simulink model "Residential_grid8"  (R2026a)
settings: Solver=VariableStepAuto  StopTime=365*24*3600
undefined symbols (not defined in the file): evCharge, load1, load2, load3, load4, load5, Solar, Wind
libraries: fl_lib x139, nesl_utility x68
(part 2 of 3)

== system Residential_grid8/Battery 5 ==
  1-D Lookup Table1 : Lookup_n-D  NumberOfTableDimensions=1  BreakpointsForDimension1=[0;0.0001;0.00025000000000000001;0.00040000000000000002;0.0007000000000000001;0.001;0.0015;0.0023;0.0040000000000000001;0.0060000000000000001;0.007000000000000001;0.0080000000000000002;0.0089999999999999993;0.0094999999999999998;0.0097999999999999997;0.0099500000000000005;0.01]  Table=[0;1;2.7000000000000002;2.9500000000000002;3.1000000000000001;3.2000000000000002;3.2400000000000002;3.2599999999999998;3.2799999999999998;3.2999999999999998;3.3399999999999999;3.3500000000000001;3.3700000000000001;3.3900000000000001;3.4500000000000002;3.6000000000000001;3.8000000000000003]  InternalRulePriority=Speed  RndMeth=Simplest
  Bus Creator : BusCreator  Inputs=3
  Capacitor : fl_lib/Electrical/Electrical Elements/Capacitor  c=3.6e5*C_batt F  r=0 Ohm  g=0 1/Ohm  i_specify=off  i_priority=None  i=0 A  i_nominal_specify=off  i_nominal_value=1  i_nominal_unit=A  v_specify=off  v_priority=None  v=0 V  v_nominal_specify=off  v_nominal_value=1  v_nominal_unit=V  vc_specify=on  vc_priority=High  vc=SOC_Initial/10000 V  vc_nominal_specify=off  vc_nominal_value=1  vc_nominal_unit=V
  Controlled Voltage Source1 : fl_lib/Electrical/Electrical Sources/Controlled Voltage Source
  Current Sensor : fl_lib/Electrical/Electrical Sensors/Current Sensor
  Gain : Gain  Gain=Cell
  Memory : Memory
  PS-Simulink Converter : nesl_utility/PS-Simulink Converter  PhysicalDomain=network_engine_domain  SubClassName=ps_output  LeftPortType=input  RightPortType=output  PseudoPeriodic=off  Frequencies=[]  VectorFormat=inherit  Unit=inherit  AffineConversion=off
  PS-Simulink Converter1 : nesl_utility/PS-Simulink Converter  PhysicalDomain=network_engine_domain  SubClassName=ps_output  LeftPortType=input  RightPortType=output  PseudoPeriodic=off  Frequencies=[]  VectorFormat=inherit  Unit=inherit  AffineConversion=off
  PS-Simulink Converter2 : nesl_utility/PS-Simulink Converter  PhysicalDomain=network_engine_domain  SubClassName=ps_output  LeftPortType=input  RightPortType=output  PseudoPeriodic=off  Frequencies=[]  VectorFormat=inherit  Unit=inherit  AffineConversion=off
  Product1 : Product
  Resistor : fl_lib/Electrical/Electrical Elements/Resistor  R=1e-3*R_int*Cell/C_batt Ohm  i_specify=off  i_priority=None  i=0 A  i_nominal_specify=off  i_nominal_value=1  i_nominal_unit=A  v_specify=off  v_priority=None  v=0 V  v_nominal_specify=off  v_nominal_value=1  v_nominal_unit=V
  Simulink-PS Converter : nesl_utility/Simulink-PS Converter  PhysicalDomain=network_engine_domain  SubClassName=ps_input  LeftPortType=input  RightPortType=output  PseudoPeriodic=off  Frequencies=[]  NoiseDistribution=none  NoiseParameters=[]  Unit=1  AffineConversion=off  FilteringAndDerivatives=provide  SimscapeFilterOrder=1  InputFilterTimeConstant=0.001  UdotUserProvided=0
  Voltage Sensor : fl_lib/Electrical/Electrical Sensors/Voltage Sensor
  Voltage Sensor1 : fl_lib/Electrical/Electrical Sensors/Voltage Sensor
  + : PMIOPort  Side=Right
  - : PMIOPort  Port=2  Side=Right
  Comp. : Outport
  wires:
  PS-Simulink Converter2/1 -> Product1/1, Bus Creator/2  "IBatt"
  PS-Simulink Converter1/1 -> Bus Creator/3, Product1/2  "VBatt"
  Product1/1 -> Bus Creator/1  "Pbatt5"
  Bus Creator/1 -> Comp./1
  PS-Simulink Converter/1 -> 1-D Lookup Table1/1
  Memory/1 -> Simulink-PS Converter/1
  Gain/1 -> Memory/1
  1-D Lookup Table1/1 -> Gain/1
  connections:
  Voltage Sensor/LConn1 -- Controlled Voltage Source1/RConn2 -- Capacitor/LConn1
  Capacitor/RConn1 -- Voltage Sensor/RConn2 -- -/RConn1 -- Voltage Sensor1/RConn2
  Voltage Sensor1/LConn1 -- +/RConn1 -- Current Sensor/RConn2
  Current Sensor/LConn1 -- Resistor/RConn1
  PS-Simulink Converter/LConn1 -- Voltage Sensor/RConn1
  Controlled Voltage Source1/LConn1 -- Resistor/LConn1
  PS-Simulink Converter1/LConn1 -- Voltage Sensor1/RConn1
  PS-Simulink Converter2/LConn1 -- Current Sensor/RConn1
  Simulink-PS Converter/RConn1 -- Controlled Voltage Source1/RConn1

== system Residential_grid8/Cable 0 ==
  Resistor : fl_lib/Electrical/Electrical Elements/Resistor  R=intR/1000*L Ohm  i_specify=off  i_priority=None  i=0 A  i_nominal_specify=off  i_nominal_value=1  i_nominal_unit=A  v_specify=off  v_priority=None  v=0 V  v_nominal_specify=off  v_nominal_value=1  v_nominal_unit=V
  Resistor1 : fl_lib/Electrical/Electrical Elements/Resistor  R=intR/1000*L Ohm  i_specify=off  i_priority=None  i=0 A  i_nominal_specify=off  i_nominal_value=1  i_nominal_unit=A  v_specify=off  v_priority=None  v=0 V  v_nominal_specify=off  v_nominal_value=1  v_nominal_unit=V
  Series RLC Branch1 : PMIOPort  Side=Left
  Series RLC Branch2 : PMIOPort  Port=2  Side=Right
  Series RLC Branch3 : PMIOPort  Port=3  Side=Left
  Series RLC Branch4 : PMIOPort  Port=4  Side=Right
  connections:
  Series RLC Branch3/RConn1 -- Resistor1/LConn1
  Series RLC Branch2/RConn1 -- Resistor/RConn1
  Series RLC Branch1/RConn1 -- Resistor/LConn1
  Series RLC Branch4/RConn1 -- Resistor1/RConn1

== system Residential_grid8/Cable 1 ==
  Resistor : fl_lib/Electrical/Electrical Elements/Resistor  R=intR/1000*L Ohm  i_specify=off  i_priority=None  i=0 A  i_nominal_specify=off  i_nominal_value=1  i_nominal_unit=A  v_specify=off  v_priority=None  v=0 V  v_nominal_specify=off  v_nominal_value=1  v_nominal_unit=V
  Resistor1 : fl_lib/Electrical/Electrical Elements/Resistor  R=intR/1000*L Ohm  i_specify=off  i_priority=None  i=0 A  i_nominal_specify=off  i_nominal_value=1  i_nominal_unit=A  v_specify=off  v_priority=None  v=0 V  v_nominal_specify=off  v_nominal_value=1  v_nominal_unit=V
  Series RLC Branch1 : PMIOPort  Side=Left
  Series RLC Branch2 : PMIOPort  Port=2  Side=Right
  Series RLC Branch3 : PMIOPort  Port=3  Side=Left
  Series RLC Branch4 : PMIOPort  Port=4  Side=Right
  connections:
  Series RLC Branch3/RConn1 -- Resistor1/LConn1
  Series RLC Branch2/RConn1 -- Resistor/RConn1
  Series RLC Branch1/RConn1 -- Resistor/LConn1
  Series RLC Branch4/RConn1 -- Resistor1/RConn1

== system Residential_grid8/Cable 1-1 ==
  Resistor : fl_lib/Electrical/Electrical Elements/Resistor  R=intR/1000*L Ohm  i_specify=off  i_priority=None  i=0 A  i_nominal_specify=off  i_nominal_value=1  i_nominal_unit=A  v_specify=off  v_priority=None  v=0 V  v_nominal_specify=off  v_nominal_value=1  v_nominal_unit=V
  Resistor1 : fl_lib/Electrical/Electrical Elements/Resistor  R=intR/1000*L Ohm  i_specify=off  i_priority=None  i=0 A  i_nominal_specify=off  i_nominal_value=1  i_nominal_unit=A  v_specify=off  v_priority=None  v=0 V  v_nominal_specify=off  v_nominal_value=1  v_nominal_unit=V
  Series RLC Branch1 : PMIOPort  Side=Left
  Series RLC Branch2 : PMIOPort  Port=2  Side=Right
  Series RLC Branch3 : PMIOPort  Port=3  Side=Left
  Series RLC Branch4 : PMIOPort  Port=4  Side=Right
  connections:
  Series RLC Branch3/RConn1 -- Resistor1/LConn1
  Series RLC Branch2/RConn1 -- Resistor/RConn1
  Series RLC Branch1/RConn1 -- Resistor/LConn1
  Series RLC Branch4/RConn1 -- Resistor1/RConn1

== system Residential_grid8/Cable 1-2 ==
  Resistor : fl_lib/Electrical/Electrical Elements/Resistor  R=intR/1000*L Ohm  i_specify=off  i_priority=None  i=0 A  i_nominal_specify=off  i_nominal_value=1  i_nominal_unit=A  v_specify=off  v_priority=None  v=0 V  v_nominal_specify=off  v_nominal_value=1  v_nominal_unit=V
  Resistor1 : fl_lib/Electrical/Electrical Elements/Resistor  R=intR/1000*L Ohm  i_specify=off  i_priority=None  i=0 A  i_nominal_specify=off  i_nominal_value=1  i_nominal_unit=A  v_specify=off  v_priority=None  v=0 V  v_nominal_specify=off  v_nominal_value=1  v_nominal_unit=V
  Series RLC Branch1 : PMIOPort  Side=Left
  Series RLC Branch2 : PMIOPort  Port=2  Side=Right
  Series RLC Branch3 : PMIOPort  Port=3  Side=Left
  Series RLC Branch4 : PMIOPort  Port=4  Side=Right
  connections:
  Series RLC Branch3/RConn1 -- Resistor1/LConn1
  Series RLC Branch2/RConn1 -- Resistor/RConn1
  Series RLC Branch1/RConn1 -- Resistor/LConn1
  Series RLC Branch4/RConn1 -- Resistor1/RConn1

== system Residential_grid8/Cable 1-3 ==
  Resistor : fl_lib/Electrical/Electrical Elements/Resistor  R=intR/1000*L Ohm  i_specify=off  i_priority=None  i=0 A  i_nominal_specify=off  i_nominal_value=1  i_nominal_unit=A  v_specify=off  v_priority=None  v=0 V  v_nominal_specify=off  v_nominal_value=1  v_nominal_unit=V
  Resistor1 : fl_lib/Electrical/Electrical Elements/Resistor  R=intR/1000*L Ohm  i_specify=off  i_priority=None  i=0 A  i_nominal_specify=off  i_nominal_value=1  i_nominal_unit=A  v_specify=off  v_priority=None  v=0 V  v_nominal_specify=off  v_nominal_value=1  v_nominal_unit=V
  Series RLC Branch1 : PMIOPort  Side=Left
  Series RLC Branch2 : PMIOPort  Port=2  Side=Right
  Series RLC Branch3 : PMIOPort  Port=3  Side=Left
  Series RLC Branch4 : PMIOPort  Port=4  Side=Right
  connections:
  Series RLC Branch3/RConn1 -- Resistor1/LConn1
  Series RLC Branch2/RConn1 -- Resistor/RConn1
  Series RLC Branch1/RConn1 -- Resistor/LConn1
  Series RLC Branch4/RConn1 -- Resistor1/RConn1

== system Residential_grid8/Cable 2 ==
  Resistor : fl_lib/Electrical/Electrical Elements/Resistor  R=intR/1000*L Ohm  i_specify=off  i_priority=None  i=0 A  i_nominal_specify=off  i_nominal_value=1  i_nominal_unit=A  v_specify=off  v_priority=None  v=0 V  v_nominal_specify=off  v_nominal_value=1  v_nominal_unit=V
  Resistor1 : fl_lib/Electrical/Electrical Elements/Resistor  R=intR/1000*L Ohm  i_specify=off  i_priority=None  i=0 A  i_nominal_specify=off  i_nominal_value=1  i_nominal_unit=A  v_specify=off  v_priority=None  v=0 V  v_nominal_specify=off  v_nominal_value=1  v_nominal_unit=V
  Series RLC Branch1 : PMIOPort  Side=Left
  Series RLC Branch2 : PMIOPort  Port=2  Side=Right
  Series RLC Branch3 : PMIOPort  Port=3  Side=Left
  Series RLC Branch4 : PMIOPort  Port=4  Side=Right
  connections:
  Series RLC Branch3/RConn1 -- Resistor1/LConn1
  Series RLC Branch2/RConn1 -- Resistor/RConn1
  Series RLC Branch1/RConn1 -- Resistor/LConn1
  Series RLC Branch4/RConn1 -- Resistor1/RConn1

== system Residential_grid8/Cable 2-1 ==
  Resistor : fl_lib/Electrical/Electrical Elements/Resistor  R=intR/1000*L Ohm  i_specify=off  i_priority=None  i=0 A  i_nominal_specify=off  i_nominal_value=1  i_nominal_unit=A  v_specify=off  v_priority=None  v=0 V  v_nominal_specify=off  v_nominal_value=1  v_nominal_unit=V
  Resistor1 : fl_lib/Electrical/Electrical Elements/Resistor  R=intR/1000*L Ohm  i_specify=off  i_priority=None  i=0 A  i_nominal_specify=off  i_nominal_value=1  i_nominal_unit=A  v_specify=off  v_priority=None  v=0 V  v_nominal_specify=off  v_nominal_value=1  v_nominal_unit=V
  Series RLC Branch1 : PMIOPort  Side=Left
  Series RLC Branch2 : PMIOPort  Port=2  Side=Right
  Series RLC Branch3 : PMIOPort  Port=3  Side=Left
  Series RLC Branch4 : PMIOPort  Port=4  Side=Right
  connections:
  Series RLC Branch3/RConn1 -- Resistor1/LConn1
  Series RLC Branch2/RConn1 -- Resistor/RConn1
  Series RLC Branch1/RConn1 -- Resistor/LConn1
  Series RLC Branch4/RConn1 -- Resistor1/RConn1

== system Residential_grid8/Cable 2-2 ==
  Resistor : fl_lib/Electrical/Electrical Elements/Resistor  R=intR/1000*L Ohm  i_specify=off  i_priority=None  i=0 A  i_nominal_specify=off  i_nominal_value=1  i_nominal_unit=A  v_specify=off  v_priority=None  v=0 V  v_nominal_specify=off  v_nominal_value=1  v_nominal_unit=V
  Resistor1 : fl_lib/Electrical/Electrical Elements/Resistor  R=intR/1000*L Ohm  i_specify=off  i_priority=None  i=0 A  i_nominal_specify=off  i_nominal_value=1  i_nominal_unit=A  v_specify=off  v_priority=None  v=0 V  v_nominal_specify=off  v_nominal_value=1  v_nominal_unit=V
  Series RLC Branch1 : PMIOPort  Side=Left
  Series RLC Branch2 : PMIOPort  Port=2  Side=Right
  Series RLC Branch3 : PMIOPort  Port=3  Side=Left
  Series RLC Branch4 : PMIOPort  Port=4  Side=Right
  connections:
  Series RLC Branch3/RConn1 -- Resistor1/LConn1
  Series RLC Branch2/RConn1 -- Resistor/RConn1
  Series RLC Branch1/RConn1 -- Resistor/LConn1
  Series RLC Branch4/RConn1 -- Resistor1/RConn1

== system Residential_grid8/Cable 2-3 ==
  Resistor : fl_lib/Electrical/Electrical Elements/Resistor  R=intR/1000*L Ohm  i_specify=off  i_priority=None  i=0 A  i_nominal_specify=off  i_nominal_value=1  i_nominal_unit=A  v_specify=off  v_priority=None  v=0 V  v_nominal_specify=off  v_nominal_value=1  v_nominal_unit=V
  Resistor1 : fl_lib/Electrical/Electrical Elements/Resistor  R=intR/1000*L Ohm  i_specify=off  i_priority=None  i=0 A  i_nominal_specify=off  i_nominal_value=1  i_nominal_unit=A  v_specify=off  v_priority=None  v=0 V  v_nominal_specify=off  v_nominal_value=1  v_nominal_unit=V
  Series RLC Branch1 : PMIOPort  Side=Left
  Series RLC Branch2 : PMIOPort  Port=2  Side=Right
  Series RLC Branch3 : PMIOPort  Port=3  Side=Left
  Series RLC Branch4 : PMIOPort  Port=4  Side=Right
  connections:
  Series RLC Branch3/RConn1 -- Resistor1/LConn1
  Series RLC Branch2/RConn1 -- Resistor/RConn1
  Series RLC Branch1/RConn1 -- Resistor/LConn1
  Series RLC Branch4/RConn1 -- Resistor1/RConn1

== system Residential_grid8/Cable 3 ==
  Resistor : fl_lib/Electrical/Electrical Elements/Resistor  R=intR/1000*L Ohm  i_specify=off  i_priority=None  i=0 A  i_nominal_specify=off  i_nominal_value=1  i_nominal_unit=A  v_specify=off  v_priority=None  v=0 V  v_nominal_specify=off  v_nominal_value=1  v_nominal_unit=V
  Resistor1 : fl_lib/Electrical/Electrical Elements/Resistor  R=intR/1000*L Ohm  i_specify=off  i_priority=None  i=0 A  i_nominal_specify=off  i_nominal_value=1  i_nominal_unit=A  v_specify=off  v_priority=None  v=0 V  v_nominal_specify=off  v_nominal_value=1  v_nominal_unit=V
  Series RLC Branch1 : PMIOPort  Side=Left
  Series RLC Branch2 : PMIOPort  Port=2  Side=Right
  Series RLC Branch3 : PMIOPort  Port=3  Side=Left
  Series RLC Branch4 : PMIOPort  Port=4  Side=Right
  connections:
  Series RLC Branch3/RConn1 -- Resistor1/LConn1
  Series RLC Branch2/RConn1 -- Resistor/RConn1
  Series RLC Branch1/RConn1 -- Resistor/LConn1
  Series RLC Branch4/RConn1 -- Resistor1/RConn1

== system Residential_grid8/Cable 3-1 ==
  Resistor : fl_lib/Electrical/Electrical Elements/Resistor  R=intR/1000*L Ohm  i_specify=off  i_priority=None  i=0 A  i_nominal_specify=off  i_nominal_value=1  i_nominal_unit=A  v_specify=off  v_priority=None  v=0 V  v_nominal_specify=off  v_nominal_value=1  v_nominal_unit=V
  Resistor1 : fl_lib/Electrical/Electrical Elements/Resistor  R=intR/1000*L Ohm  i_specify=off  i_priority=None  i=0 A  i_nominal_specify=off  i_nominal_value=1  i_nominal_unit=A  v_specify=off  v_priority=None  v=0 V  v_nominal_specify=off  v_nominal_value=1  v_nominal_unit=V
  Series RLC Branch1 : PMIOPort  Side=Left
  Series RLC Branch2 : PMIOPort  Port=2  Side=Right
  Series RLC Branch3 : PMIOPort  Port=3  Side=Left
  Series RLC Branch4 : PMIOPort  Port=4  Side=Right
  connections:
  Series RLC Branch3/RConn1 -- Resistor1/LConn1
  Series RLC Branch2/RConn1 -- Resistor/RConn1
  Series RLC Branch1/RConn1 -- Resistor/LConn1
  Series RLC Branch4/RConn1 -- Resistor1/RConn1

== system Residential_grid8/Cable 3-2 ==
  Resistor : fl_lib/Electrical/Electrical Elements/Resistor  R=intR/1000*L Ohm  i_specify=off  i_priority=None  i=0 A  i_nominal_specify=off  i_nominal_value=1  i_nominal_unit=A  v_specify=off  v_priority=None  v=0 V  v_nominal_specify=off  v_nominal_value=1  v_nominal_unit=V
  Resistor1 : fl_lib/Electrical/Electrical Elements/Resistor  R=intR/1000*L Ohm  i_specify=off  i_priority=None  i=0 A  i_nominal_specify=off  i_nominal_value=1  i_nominal_unit=A  v_specify=off  v_priority=None  v=0 V  v_nominal_specify=off  v_nominal_value=1  v_nominal_unit=V
  Series RLC Branch1 : PMIOPort  Side=Left
  Series RLC Branch2 : PMIOPort  Port=2  Side=Right
  Series RLC Branch3 : PMIOPort  Port=3  Side=Left
  Series RLC Branch4 : PMIOPort  Port=4  Side=Right
  connections:
  Series RLC Branch3/RConn1 -- Resistor1/LConn1
  Series RLC Branch2/RConn1 -- Resistor/RConn1
  Series RLC Branch1/RConn1 -- Resistor/LConn1
  Series RLC Branch4/RConn1 -- Resistor1/RConn1

== system Residential_grid8/Cable 3-3 ==
  Resistor : fl_lib/Electrical/Electrical Elements/Resistor  R=intR/1000*L Ohm  i_specify=off  i_priority=None  i=0 A  i_nominal_specify=off  i_nominal_value=1  i_nominal_unit=A  v_specify=off  v_priority=None  v=0 V  v_nominal_specify=off  v_nominal_value=1  v_nominal_unit=V
  Resistor1 : fl_lib/Electrical/Electrical Elements/Resistor  R=intR/1000*L Ohm  i_specify=off  i_priority=None  i=0 A  i_nominal_specify=off  i_nominal_value=1  i_nominal_unit=A  v_specify=off  v_priority=None  v=0 V  v_nominal_specify=off  v_nominal_value=1  v_nominal_unit=V
  Series RLC Branch1 : PMIOPort  Side=Left
  Series RLC Branch2 : PMIOPort  Port=2  Side=Right
  Series RLC Branch3 : PMIOPort  Port=3  Side=Left
  Series RLC Branch4 : PMIOPort  Port=4  Side=Right
  connections:
  Series RLC Branch3/RConn1 -- Resistor1/LConn1
  Series RLC Branch2/RConn1 -- Resistor/RConn1
  Series RLC Branch1/RConn1 -- Resistor/LConn1
  Series RLC Branch4/RConn1 -- Resistor1/RConn1

== system Residential_grid8/Cable 3-4 ==
  Resistor : fl_lib/Electrical/Electrical Elements/Resistor  R=intR/1000*L Ohm  i_specify=off  i_priority=None  i=0 A  i_nominal_specify=off  i_nominal_value=1  i_nominal_unit=A  v_specify=off  v_priority=None  v=0 V  v_nominal_specify=off  v_nominal_value=1  v_nominal_unit=V
  Resistor1 : fl_lib/Electrical/Electrical Elements/Resistor  R=intR/1000*L Ohm  i_specify=off  i_priority=None  i=0 A  i_nominal_specify=off  i_nominal_value=1  i_nominal_unit=A  v_specify=off  v_priority=None  v=0 V  v_nominal_specify=off  v_nominal_value=1  v_nominal_unit=V
  Series RLC Branch1 : PMIOPort  Side=Left
  Series RLC Branch2 : PMIOPort  Port=2  Side=Right
  Series RLC Branch3 : PMIOPort  Port=3  Side=Left
  Series RLC Branch4 : PMIOPort  Port=4  Side=Right
  connections:
  Series RLC Branch3/RConn1 -- Resistor1/LConn1
  Series RLC Branch2/RConn1 -- Resistor/RConn1
  Series RLC Branch1/RConn1 -- Resistor/LConn1
  Series RLC Branch4/RConn1 -- Resistor1/RConn1

== system Residential_grid8/Cable 4 ==
  Resistor : fl_lib/Electrical/Electrical Elements/Resistor  R=intR/1000*L Ohm  i_specify=off  i_priority=None  i=0 A  i_nominal_specify=off  i_nominal_value=1  i_nominal_unit=A  v_specify=off  v_priority=None  v=0 V  v_nominal_specify=off  v_nominal_value=1  v_nominal_unit=V
  Resistor1 : fl_lib/Electrical/Electrical Elements/Resistor  R=intR/1000*L Ohm  i_specify=off  i_priority=None  i=0 A  i_nominal_specify=off  i_nominal_value=1  i_nominal_unit=A  v_specify=off  v_priority=None  v=0 V  v_nominal_specify=off  v_nominal_value=1  v_nominal_unit=V
  Series RLC Branch1 : PMIOPort  Side=Left
  Series RLC Branch2 : PMIOPort  Port=2  Side=Right
  Series RLC Branch3 : PMIOPort  Port=3  Side=Left
  Series RLC Branch4 : PMIOPort  Port=4  Side=Right
  connections:
  Series RLC Branch3/RConn1 -- Resistor1/LConn1
  Series RLC Branch2/RConn1 -- Resistor/RConn1
  Series RLC Branch1/RConn1 -- Resistor/LConn1
  Series RLC Branch4/RConn1 -- Resistor1/RConn1

== system Residential_grid8/Cable 4-1 ==
  Resistor : fl_lib/Electrical/Electrical Elements/Resistor  R=intR/1000*L Ohm  i_specify=off  i_priority=None  i=0 A  i_nominal_specify=off  i_nominal_value=1  i_nominal_unit=A  v_specify=off  v_priority=None  v=0 V  v_nominal_specify=off  v_nominal_value=1  v_nominal_unit=V
  Resistor1 : fl_lib/Electrical/Electrical Elements/Resistor  R=intR/1000*L Ohm  i_specify=off  i_priority=None  i=0 A  i_nominal_specify=off  i_nominal_value=1  i_nominal_unit=A  v_specify=off  v_priority=None  v=0 V  v_nominal_specify=off  v_nominal_value=1  v_nominal_unit=V
  Series RLC Branch1 : PMIOPort  Side=Left
  Series RLC Branch2 : PMIOPort  Port=2  Side=Right
  Series RLC Branch3 : PMIOPort  Port=3  Side=Left
  Series RLC Branch4 : PMIOPort  Port=4  Side=Right
  connections:
  Series RLC Branch3/RConn1 -- Resistor1/LConn1
  Series RLC Branch2/RConn1 -- Resistor/RConn1
  Series RLC Branch1/RConn1 -- Resistor/LConn1
  Series RLC Branch4/RConn1 -- Resistor1/RConn1

== system Residential_grid8/Cable 4-2 ==
  Resistor : fl_lib/Electrical/Electrical Elements/Resistor  R=intR/1000*L Ohm  i_specify=off  i_priority=None  i=0 A  i_nominal_specify=off  i_nominal_value=1  i_nominal_unit=A  v_specify=off  v_priority=None  v=0 V  v_nominal_specify=off  v_nominal_value=1  v_nominal_unit=V
  Resistor1 : fl_lib/Electrical/Electrical Elements/Resistor  R=intR/1000*L Ohm  i_specify=off  i_priority=None  i=0 A  i_nominal_specify=off  i_nominal_value=1  i_nominal_unit=A  v_specify=off  v_priority=None  v=0 V  v_nominal_specify=off  v_nominal_value=1  v_nominal_unit=V
  Series RLC Branch1 : PMIOPort  Side=Left
  Series RLC Branch2 : PMIOPort  Port=2  Side=Right
  Series RLC Branch3 : PMIOPort  Port=3  Side=Left
  Series RLC Branch4 : PMIOPort  Port=4  Side=Right
  connections:
  Series RLC Branch3/RConn1 -- Resistor1/LConn1
  Series RLC Branch2/RConn1 -- Resistor/RConn1
  Series RLC Branch1/RConn1 -- Resistor/LConn1
  Series RLC Branch4/RConn1 -- Resistor1/RConn1

== system Residential_grid8/Cable 4-3 ==
  Resistor : fl_lib/Electrical/Electrical Elements/Resistor  R=intR/1000*L Ohm  i_specify=off  i_priority=None  i=0 A  i_nominal_specify=off  i_nominal_value=1  i_nominal_unit=A  v_specify=off  v_priority=None  v=0 V  v_nominal_specify=off  v_nominal_value=1  v_nominal_unit=V
  Resistor1 : fl_lib/Electrical/Electrical Elements/Resistor  R=intR/1000*L Ohm  i_specify=off  i_priority=None  i=0 A  i_nominal_specify=off  i_nominal_value=1  i_nominal_unit=A  v_specify=off  v_priority=None  v=0 V  v_nominal_specify=off  v_nominal_value=1  v_nominal_unit=V
  Series RLC Branch1 : PMIOPort  Side=Left
  Series RLC Branch2 : PMIOPort  Port=2  Side=Right
  Series RLC Branch3 : PMIOPort  Port=3  Side=Left
  Series RLC Branch4 : PMIOPort  Port=4  Side=Right
  connections:
  Series RLC Branch3/RConn1 -- Resistor1/LConn1
  Series RLC Branch2/RConn1 -- Resistor/RConn1
  Series RLC Branch1/RConn1 -- Resistor/LConn1
  Series RLC Branch4/RConn1 -- Resistor1/RConn1

== system Residential_grid8/Cable 5 ==
  Resistor : fl_lib/Electrical/Electrical Elements/Resistor  R=intR/1000*L Ohm  i_specify=off  i_priority=None  i=0 A  i_nominal_specify=off  i_nominal_value=1  i_nominal_unit=A  v_specify=off  v_priority=None  v=0 V  v_nominal_specify=off  v_nominal_value=1  v_nominal_unit=V
  Resistor1 : fl_lib/Electrical/Electrical Elements/Resistor  R=intR/1000*L Ohm  i_specify=off  i_priority=None  i=0 A  i_nominal_specify=off  i_nominal_value=1  i_nominal_unit=A  v_specify=off  v_priority=None  v=0 V  v_nominal_specify=off  v_nominal_value=1  v_nominal_unit=V
  Series RLC Branch1 : PMIOPort  Side=Left
  Series RLC Branch2 : PMIOPort  Port=2  Side=Right
  Series RLC Branch3 : PMIOPort  Port=3  Side=Left
  Series RLC Branch4 : PMIOPort  Port=4  Side=Right
  connections:
  Series RLC Branch3/RConn1 -- Resistor1/LConn1
  Series RLC Branch2/RConn1 -- Resistor/RConn1
  Series RLC Branch1/RConn1 -- Resistor/LConn1
  Series RLC Branch4/RConn1 -- Resistor1/RConn1

== system Residential_grid8/Cable 5-1 ==
  Resistor : fl_lib/Electrical/Electrical Elements/Resistor  R=intR/1000*L Ohm  i_specify=off  i_priority=None  i=0 A  i_nominal_specify=off  i_nominal_value=1  i_nominal_unit=A  v_specify=off  v_priority=None  v=0 V  v_nominal_specify=off  v_nominal_value=1  v_nominal_unit=V
  Resistor1 : fl_lib/Electrical/Electrical Elements/Resistor  R=intR/1000*L Ohm  i_specify=off  i_priority=None  i=0 A  i_nominal_specify=off  i_nominal_value=1  i_nominal_unit=A  v_specify=off  v_priority=None  v=0 V  v_nominal_specify=off  v_nominal_value=1  v_nominal_unit=V
  Series RLC Branch1 : PMIOPort  Side=Left
  Series RLC Branch2 : PMIOPort  Port=2  Side=Right
  Series RLC Branch3 : PMIOPort  Port=3  Side=Left
  Series RLC Branch4 : PMIOPort  Port=4  Side=Right
  connections:
  Series RLC Branch3/RConn1 -- Resistor1/LConn1
  Series RLC Branch2/RConn1 -- Resistor/RConn1
  Series RLC Branch1/RConn1 -- Resistor/LConn1
  Series RLC Branch4/RConn1 -- Resistor1/RConn1

== system Residential_grid8/Cable 5-2 ==
  Resistor : fl_lib/Electrical/Electrical Elements/Resistor  R=intR/1000*L Ohm  i_specify=off  i_priority=None  i=0 A  i_nominal_specify=off  i_nominal_value=1  i_nominal_unit=A  v_specify=off  v_priority=None  v=0 V  v_nominal_specify=off  v_nominal_value=1  v_nominal_unit=V
  Resistor1 : fl_lib/Electrical/Electrical Elements/Resistor  R=intR/1000*L Ohm  i_specify=off  i_priority=None  i=0 A  i_nominal_specify=off  i_nominal_value=1  i_nominal_unit=A  v_specify=off  v_priority=None  v=0 V  v_nominal_specify=off  v_nominal_value=1  v_nominal_unit=V
  Series RLC Branch1 : PMIOPort  Side=Left
  Series RLC Branch2 : PMIOPort  Port=2  Side=Right
  Series RLC Branch3 : PMIOPort  Port=3  Side=Left
  Series RLC Branch4 : PMIOPort  Port=4  Side=Right
  connections:
  Series RLC Branch3/RConn1 -- Resistor1/LConn1
  Series RLC Branch2/RConn1 -- Resistor/RConn1
  Series RLC Branch1/RConn1 -- Resistor/LConn1
  Series RLC Branch4/RConn1 -- Resistor1/RConn1

== system Residential_grid8/Cable 5-3 ==
  Resistor : fl_lib/Electrical/Electrical Elements/Resistor  R=intR/1000*L Ohm  i_specify=off  i_priority=None  i=0 A  i_nominal_specify=off  i_nominal_value=1  i_nominal_unit=A  v_specify=off  v_priority=None  v=0 V  v_nominal_specify=off  v_nominal_value=1  v_nominal_unit=V
  Resistor1 : fl_lib/Electrical/Electrical Elements/Resistor  R=intR/1000*L Ohm  i_specify=off  i_priority=None  i=0 A  i_nominal_specify=off  i_nominal_value=1  i_nominal_unit=A  v_specify=off  v_priority=None  v=0 V  v_nominal_specify=off  v_nominal_value=1  v_nominal_unit=V
  Series RLC Branch1 : PMIOPort  Side=Left
  Series RLC Branch2 : PMIOPort  Port=2  Side=Right
  Series RLC Branch3 : PMIOPort  Port=3  Side=Left
  Series RLC Branch4 : PMIOPort  Port=4  Side=Right
  connections:
  Series RLC Branch3/RConn1 -- Resistor1/LConn1
  Series RLC Branch2/RConn1 -- Resistor/RConn1
  Series RLC Branch1/RConn1 -- Resistor/LConn1
  Series RLC Branch4/RConn1 -- Resistor1/RConn1

== system Residential_grid8/Cable 6 ==
  Resistor : fl_lib/Electrical/Electrical Elements/Resistor  R=intR/1000*L Ohm  i_specify=off  i_priority=None  i=0 A  i_nominal_specify=off  i_nominal_value=1  i_nominal_unit=A  v_specify=off  v_priority=None  v=0 V  v_nominal_specify=off  v_nominal_value=1  v_nominal_unit=V
  Resistor1 : fl_lib/Electrical/Electrical Elements/Resistor  R=intR/1000*L Ohm  i_specify=off  i_priority=None  i=0 A  i_nominal_specify=off  i_nominal_value=1  i_nominal_unit=A  v_specify=off  v_priority=None  v=0 V  v_nominal_specify=off  v_nominal_value=1  v_nominal_unit=V
  Series RLC Branch1 : PMIOPort  Side=Left
  Series RLC Branch2 : PMIOPort  Port=2  Side=Right
  Series RLC Branch3 : PMIOPort  Port=3  Side=Left
  Series RLC Branch4 : PMIOPort  Port=4  Side=Right
  connections:
  Series RLC Branch3/RConn1 -- Resistor1/LConn1
  Series RLC Branch2/RConn1 -- Resistor/RConn1
  Series RLC Branch1/RConn1 -- Resistor/LConn1
  Series RLC Branch4/RConn1 -- Resistor1/RConn1

== system Residential_grid8/EV charging ==
  Clock : Clock
  Controlled Current Source1 : fl_lib/Electrical/Electrical Sources/Controlled Current Source
  Current Sensor : fl_lib/Electrical/Electrical Sensors/Current Sensor
  Divide : Product  Inputs=*/
  Memory1 : Memory
  PS-Simulink Converter : nesl_utility/PS-Simulink Converter  PhysicalDomain=network_engine_domain  SubClassName=ps_output  LeftPortType=input  RightPortType=output  PseudoPeriodic=off  Frequencies=[]  VectorFormat=inherit  Unit=inherit  AffineConversion=off
  PS-Simulink Converter1 : nesl_utility/PS-Simulink Converter  PhysicalDomain=network_engine_domain  SubClassName=ps_output  LeftPortType=input  RightPortType=output  PseudoPeriodic=off  Frequencies=[]  VectorFormat=inherit  Unit=inherit  AffineConversion=off
  Power consumption : Lookup_n-D  NumberOfTableDimensions=1  BreakpointsForDimension1=timestep  BeginIndexSearchUsingPreviousIndexResult=on  Table=data  InternalRulePriority=Speed  RndMeth=Simplest
  Product4 : Product
  Resistor1 : fl_lib/Electrical/Electrical Elements/Resistor  R=1e10 Ohm  i_specify=off  i_priority=None  i=0 A  i_nominal_specify=off  i_nominal_value=1  i_nominal_unit=A  v_specify=off  v_priority=None  v=0 V  v_nominal_specify=off  v_nominal_value=1  v_nominal_unit=V
  Simulink-PS Converter : nesl_utility/Simulink-PS Converter  PhysicalDomain=network_engine_domain  SubClassName=ps_input  LeftPortType=input  RightPortType=output  PseudoPeriodic=off  Frequencies=[]  NoiseDistribution=none  NoiseParameters=[]  Unit=1  AffineConversion=off  FilteringAndDerivatives=provide  SimscapeFilterOrder=1  InputFilterTimeConstant=0.001  UdotUserProvided=0
  Voltage Sensor : fl_lib/Electrical/Electrical Sensors/Voltage Sensor
  +190 V : PMIOPort  Side=Right
  -190 V : PMIOPort  Port=2  Side=Right
  P : Outport
  V : Outport  Port=2
  wires:
  Clock/1 -> Power consumption/1
  Power consumption/1 -> Divide/1
  PS-Simulink Converter1/1 -> V/1, Product4/2, Divide/2  "V_Load"
  Product4/1 -> P/1
  Divide/1 -> Memory1/1
  Memory1/1 -> Simulink-PS Converter/1
  PS-Simulink Converter/1 -> Product4/1
  connections:
  Resistor1/LConn1 -- Controlled Current Source1/RConn2 -- Current Sensor/LConn1
  +190 V/RConn1 -- Voltage Sensor/LConn1 -- Current Sensor/RConn2
  -190 V/RConn1 -- Voltage Sensor/RConn2 -- Controlled Current Source1/LConn1 -- Resistor1/RConn1
  Simulink-PS Converter/RConn1 -- Controlled Current Source1/RConn1
  PS-Simulink Converter1/LConn1 -- Voltage Sensor/RConn1
  PS-Simulink Converter/LConn1 -- Current Sensor/RConn1

== system Residential_grid8/P_Grid ==
  In1 : Inport
  Bus Selector : BusSelector  OutputSignals=vbus,ibus
  Gain : Gain  Gain=-1
  Product1 : Product
  Product4 : Product
  Saturation1 : Saturate  UpperLimit=inf  LowerLimit=0
  Saturation2 : Saturate  UpperLimit=0  LowerLimit=-inf
  Out1 : Outport
  Out2 : Outport  Port=2
  wires:
  In1/1 -> Bus Selector/1
  Bus Selector/2 -> Saturation2/1, Saturation1/1  "<ibus>"
  Bus Selector/1 -> Product4/1, Product1/1  "<vbus>"
  Saturation1/1 -> Product1/2
  Saturation2/1 -> Product4/2
  Product1/1 -> Out1/1  "(Local grid)"
  Product4/1 -> Gain/1  "(Local grid)"
  Gain/1 -> Out2/1

== system Residential_grid8/Power ==
  P_grid1 : Inport
  P_grid2 : Inport  Port=2
  P_load : Inport  Port=3
  Gain1 : Gain  Gain=-1
  Integrator1 : Integrator  InitialCondition=1  LimitOutput=on  LowerSaturationLimit=0
  Integrator2 : Integrator  InitialCondition=1  LimitOutput=on  LowerSaturationLimit=0
  Integrator3 : Integrator  InitialCondition=1
  From Grid : Outport
  To Grid : Outport  Port=2
  Total Consumption : Outport  Port=3
  wires:
  Integrator1/1 -> From Grid/1  "From Grid"
  Integrator3/1 -> Total Consumption/1  "Total Consumption"
  Gain1/1 -> Integrator3/1
  P_load/1 -> Gain1/1
  P_grid1/1 -> Integrator1/1
  Integrator2/1 -> To Grid/1  "To Grid"
  P_grid2/1 -> Integrator2/1

== system Residential_grid8/Power load 1 ==
  Clock : Clock
  Controlled Current Source1 : fl_lib/Electrical/Electrical Sources/Controlled Current Source
  Current Sensor : fl_lib/Electrical/Electrical Sensors/Current Sensor
  Divide : Product  Inputs=*/
  Memory1 : Memory
  PS-Simulink Converter : nesl_utility/PS-Simulink Converter  PhysicalDomain=network_engine_domain  SubClassName=ps_output  LeftPortType=input  RightPortType=output  PseudoPeriodic=off  Frequencies=[]  VectorFormat=inherit  Unit=inherit  AffineConversion=off
  PS-Simulink Converter1 : nesl_utility/PS-Simulink Converter  PhysicalDomain=network_engine_domain  SubClassName=ps_output  LeftPortType=input  RightPortType=output  PseudoPeriodic=off  Frequencies=[]  VectorFormat=inherit  Unit=inherit  AffineConversion=off
  Power consumption : Lookup_n-D  NumberOfTableDimensions=1  BreakpointsForDimension1=timestep  BeginIndexSearchUsingPreviousIndexResult=on  Table=data  InternalRulePriority=Speed  RndMeth=Simplest
  Product4 : Product
  Resistor1 : fl_lib/Electrical/Electrical Elements/Resistor  R=1e10 Ohm  i_specify=off  i_priority=None  i=0 A  i_nominal_specify=off  i_nominal_value=1  i_nominal_unit=A  v_specify=off  v_priority=None  v=0 V  v_nominal_specify=off  v_nominal_value=1  v_nominal_unit=V
  Simulink-PS Converter : nesl_utility/Simulink-PS Converter  PhysicalDomain=network_engine_domain  SubClassName=ps_input  LeftPortType=input  RightPortType=output  PseudoPeriodic=off  Frequencies=[]  NoiseDistribution=none  NoiseParameters=[]  Unit=1  AffineConversion=off  FilteringAndDerivatives=provide  SimscapeFilterOrder=1  InputFilterTimeConstant=0.001  UdotUserProvided=0
  Voltage Sensor : fl_lib/Electrical/Electrical Sensors/Voltage Sensor
  + : PMIOPort  Side=Right
  - : PMIOPort  Port=2  Side=Right
  P : Outport
  V : Outport  Port=2
  wires:
  Clock/1 -> Power consumption/1
  Power consumption/1 -> Divide/1
  PS-Simulink Converter1/1 -> Product4/2, V/1, Divide/2  "V_Load"
  PS-Simulink Converter/1 -> Product4/1
  Product4/1 -> P/1
  Divide/1 -> Memory1/1
  Memory1/1 -> Simulink-PS Converter/1
  connections:
  Current Sensor/LConn1 -- Resistor1/LConn1 -- Controlled Current Source1/RConn2
  +/RConn1 -- Current Sensor/RConn2 -- Voltage Sensor/LConn1
  Controlled Current Source1/LConn1 -- Resistor1/RConn1 -- -/RConn1 -- Voltage Sensor/RConn2
  Simulink-PS Converter/RConn1 -- Controlled Current Source1/RConn1
  Current Sensor/RConn1 -- PS-Simulink Converter/LConn1
  PS-Simulink Converter1/LConn1 -- Voltage Sensor/RConn1

== system Residential_grid8/Power load 2 ==
  Clock : Clock
  Controlled Current Source1 : fl_lib/Electrical/Electrical Sources/Controlled Current Source
  Current Sensor : fl_lib/Electrical/Electrical Sensors/Current Sensor
  Divide : Product  Inputs=*/
  Memory1 : Memory
  PS-Simulink Converter : nesl_utility/PS-Simulink Converter  PhysicalDomain=network_engine_domain  SubClassName=ps_output  LeftPortType=input  RightPortType=output  PseudoPeriodic=off  Frequencies=[]  VectorFormat=inherit  Unit=inherit  AffineConversion=off
  PS-Simulink Converter1 : nesl_utility/PS-Simulink Converter  PhysicalDomain=network_engine_domain  SubClassName=ps_output  LeftPortType=input  RightPortType=output  PseudoPeriodic=off  Frequencies=[]  VectorFormat=inherit  Unit=inherit  AffineConversion=off
  Power consumption : Lookup_n-D  NumberOfTableDimensions=1  BreakpointsForDimension1=timestep  BeginIndexSearchUsingPreviousIndexResult=on  Table=data  InternalRulePriority=Speed  RndMeth=Simplest
  Product4 : Product
  Resistor1 : fl_lib/Electrical/Electrical Elements/Resistor  R=1e10 Ohm  i_specify=off  i_priority=None  i=0 A  i_nominal_specify=off  i_nominal_value=1  i_nominal_unit=A  v_specify=off  v_priority=None  v=0 V  v_nominal_specify=off  v_nominal_value=1  v_nominal_unit=V
  Simulink-PS Converter : nesl_utility/Simulink-PS Converter  PhysicalDomain=network_engine_domain  SubClassName=ps_input  LeftPortType=input  RightPortType=output  PseudoPeriodic=off  Frequencies=[]  NoiseDistribution=none  NoiseParameters=[]  Unit=1  AffineConversion=off  FilteringAndDerivatives=provide  SimscapeFilterOrder=1  InputFilterTimeConstant=0.001  UdotUserProvided=0
  Voltage Sensor : fl_lib/Electrical/Electrical Sensors/Voltage Sensor
  + : PMIOPort  Side=Right
  - : PMIOPort  Port=2  Side=Right
  P : Outport
  V : Outport  Port=2
  wires:
  Clock/1 -> Power consumption/1
  Power consumption/1 -> Divide/1
  PS-Simulink Converter1/1 -> Product4/2, V/1, Divide/2  "V_Load"
  PS-Simulink Converter/1 -> Product4/1
  Product4/1 -> P/1
  Divide/1 -> Memory1/1
  Memory1/1 -> Simulink-PS Converter/1
  connections:
  Current Sensor/LConn1 -- Resistor1/LConn1 -- Controlled Current Source1/RConn2
  +/RConn1 -- Current Sensor/RConn2 -- Voltage Sensor/LConn1
  Controlled Current Source1/LConn1 -- Resistor1/RConn1 -- -/RConn1 -- Voltage Sensor/RConn2
  Simulink-PS Converter/RConn1 -- Controlled Current Source1/RConn1
  Current Sensor/RConn1 -- PS-Simulink Converter/LConn1
  PS-Simulink Converter1/LConn1 -- Voltage Sensor/RConn1

== system Residential_grid8/Power load 3 ==
  Clock : Clock
  Controlled Current Source1 : fl_lib/Electrical/Electrical Sources/Controlled Current Source
  Current Sensor : fl_lib/Electrical/Electrical Sensors/Current Sensor
  Divide : Product  Inputs=*/
  Memory1 : Memory
  PS-Simulink Converter : nesl_utility/PS-Simulink Converter  PhysicalDomain=network_engine_domain  SubClassName=ps_output  LeftPortType=input  RightPortType=output  PseudoPeriodic=off  Frequencies=[]  VectorFormat=inherit  Unit=inherit  AffineConversion=off
  PS-Simulink Converter1 : nesl_utility/PS-Simulink Converter  PhysicalDomain=network_engine_domain  SubClassName=ps_output  LeftPortType=input  RightPortType=output  PseudoPeriodic=off  Frequencies=[]  VectorFormat=inherit  Unit=inherit  AffineConversion=off
  Power consumption : Lookup_n-D  NumberOfTableDimensions=1  BreakpointsForDimension1=timestep  BeginIndexSearchUsingPreviousIndexResult=on  Table=data  InternalRulePriority=Speed  RndMeth=Simplest
  Product4 : Product
  Resistor1 : fl_lib/Electrical/Electrical Elements/Resistor  R=1e10 Ohm  i_specify=off  i_priority=None  i=0 A  i_nominal_specify=off  i_nominal_value=1  i_nominal_unit=A  v_specify=off  v_priority=None  v=0 V  v_nominal_specify=off  v_nominal_value=1  v_nominal_unit=V
  Simulink-PS Converter : nesl_utility/Simulink-PS Converter  PhysicalDomain=network_engine_domain  SubClassName=ps_input  LeftPortType=input  RightPortType=output  PseudoPeriodic=off  Frequencies=[]  NoiseDistribution=none  NoiseParameters=[]  Unit=1  AffineConversion=off  FilteringAndDerivatives=provide  SimscapeFilterOrder=1  InputFilterTimeConstant=0.001  UdotUserProvided=0
  Voltage Sensor : fl_lib/Electrical/Electrical Sensors/Voltage Sensor
  + : PMIOPort  Side=Right
  - : PMIOPort  Port=2  Side=Right
  P : Outport
  V : Outport  Port=2
  wires:
  Clock/1 -> Power consumption/1
  Power consumption/1 -> Divide/1
  PS-Simulink Converter1/1 -> Product4/2, V/1, Divide/2  "V_Load"
  PS-Simulink Converter/1 -> Product4/1
  Product4/1 -> P/1
  Divide/1 -> Memory1/1
  Memory1/1 -> Simulink-PS Converter/1
  connections:
  Current Sensor/LConn1 -- Resistor1/LConn1 -- Controlled Current Source1/RConn2
  +/RConn1 -- Current Sensor/RConn2 -- Voltage Sensor/LConn1
  Controlled Current Source1/LConn1 -- Resistor1/RConn1 -- -/RConn1 -- Voltage Sensor/RConn2
  Simulink-PS Converter/RConn1 -- Controlled Current Source1/RConn1
  Current Sensor/RConn1 -- PS-Simulink Converter/LConn1
  PS-Simulink Converter1/LConn1 -- Voltage Sensor/RConn1

== system Residential_grid8/Power load 4 ==
  Clock : Clock
  Controlled Current Source1 : fl_lib/Electrical/Electrical Sources/Controlled Current Source
  Current Sensor : fl_lib/Electrical/Electrical Sensors/Current Sensor
  Divide : Product  Inputs=*/
  Memory1 : Memory
  PS-Simulink Converter : nesl_utility/PS-Simulink Converter  PhysicalDomain=network_engine_domain  SubClassName=ps_output  LeftPortType=input  RightPortType=output  PseudoPeriodic=off  Frequencies=[]  VectorFormat=inherit  Unit=inherit  AffineConversion=off
  PS-Simulink Converter1 : nesl_utility/PS-Simulink Converter  PhysicalDomain=network_engine_domain  SubClassName=ps_output  LeftPortType=input  RightPortType=output  PseudoPeriodic=off  Frequencies=[]  VectorFormat=inherit  Unit=inherit  AffineConversion=off
  Power consumption : Lookup_n-D  NumberOfTableDimensions=1  BreakpointsForDimension1=timestep  BeginIndexSearchUsingPreviousIndexResult=on  Table=data  InternalRulePriority=Speed  RndMeth=Simplest
  Product4 : Product
  Resistor1 : fl_lib/Electrical/Electrical Elements/Resistor  R=1e10 Ohm  i_specify=off  i_priority=None  i=0 A  i_nominal_specify=off  i_nominal_value=1  i_nominal_unit=A  v_specify=off  v_priority=None  v=0 V  v_nominal_specify=off  v_nominal_value=1  v_nominal_unit=V
  Simulink-PS Converter : nesl_utility/Simulink-PS Converter  PhysicalDomain=network_engine_domain  SubClassName=ps_input  LeftPortType=input  RightPortType=output  PseudoPeriodic=off  Frequencies=[]  NoiseDistribution=none  NoiseParameters=[]  Unit=1  AffineConversion=off  FilteringAndDerivatives=provide  SimscapeFilterOrder=1  InputFilterTimeConstant=0.001  UdotUserProvided=0
  Voltage Sensor : fl_lib/Electrical/Electrical Sensors/Voltage Sensor
  + : PMIOPort  Side=Right
  - : PMIOPort  Port=2  Side=Right
  P : Outport
  V : Outport  Port=2
  wires:
  Clock/1 -> Power consumption/1
  Power consumption/1 -> Divide/1
  PS-Simulink Converter1/1 -> Product4/2, V/1, Divide/2  "V_Load"
  PS-Simulink Converter/1 -> Product4/1
  Product4/1 -> P/1
  Divide/1 -> Memory1/1
  Memory1/1 -> Simulink-PS Converter/1
  connections:
  Current Sensor/LConn1 -- Resistor1/LConn1 -- Controlled Current Source1/RConn2
  +/RConn1 -- Current Sensor/RConn2 -- Voltage Sensor/LConn1
  Controlled Current Source1/LConn1 -- Resistor1/RConn1 -- -/RConn1 -- Voltage Sensor/RConn2
  Simulink-PS Converter/RConn1 -- Controlled Current Source1/RConn1
  Current Sensor/RConn1 -- PS-Simulink Converter/LConn1
  PS-Simulink Converter1/LConn1 -- Voltage Sensor/RConn1

== system Residential_grid8/Power load 5 ==
  Clock : Clock
  Controlled Current Source1 : fl_lib/Electrical/Electrical Sources/Controlled Current Source
  Current Sensor : fl_lib/Electrical/Electrical Sensors/Current Sensor
  Divide : Product  Inputs=*/
  Memory1 : Memory
  PS-Simulink Converter : nesl_utility/PS-Simulink Converter  PhysicalDomain=network_engine_domain  SubClassName=ps_output  LeftPortType=input  RightPortType=output  PseudoPeriodic=off  Frequencies=[]  VectorFormat=inherit  Unit=inherit  AffineConversion=off
  PS-Simulink Converter1 : nesl_utility/PS-Simulink Converter  PhysicalDomain=network_engine_domain  SubClassName=ps_output  LeftPortType=input  RightPortType=output  PseudoPeriodic=off  Frequencies=[]  VectorFormat=inherit  Unit=inherit  AffineConversion=off
  Power consumption : Lookup_n-D  NumberOfTableDimensions=1  BreakpointsForDimension1=timestep  BeginIndexSearchUsingPreviousIndexResult=on  Table=data  InternalRulePriority=Speed  RndMeth=Simplest
  Product4 : Product
  Resistor1 : fl_lib/Electrical/Electrical Elements/Resistor  R=1e10 Ohm  i_specify=off  i_priority=None  i=0 A  i_nominal_specify=off  i_nominal_value=1  i_nominal_unit=A  v_specify=off  v_priority=None  v=0 V  v_nominal_specify=off  v_nominal_value=1  v_nominal_unit=V
  Simulink-PS Converter : nesl_utility/Simulink-PS Converter  PhysicalDomain=network_engine_domain  SubClassName=ps_input  LeftPortType=input  RightPortType=output  PseudoPeriodic=off  Frequencies=[]  NoiseDistribution=none  NoiseParameters=[]  Unit=1  AffineConversion=off  FilteringAndDerivatives=provide  SimscapeFilterOrder=1  InputFilterTimeConstant=0.001  UdotUserProvided=0
  Voltage Sensor : fl_lib/Electrical/Electrical Sensors/Voltage Sensor
  + : PMIOPort  Side=Right
  - : PMIOPort  Port=2  Side=Right
  P : Outport
  V : Outport  Port=2
  wires:
  Clock/1 -> Power consumption/1
  Power consumption/1 -> Divide/1
  PS-Simulink Converter1/1 -> Product4/2, V/1, Divide/2  "V_Load"
  PS-Simulink Converter/1 -> Product4/1
  Product4/1 -> P/1
  Divide/1 -> Memory1/1
  Memory1/1 -> Simulink-PS Converter/1
  connections:
  Current Sensor/LConn1 -- Resistor1/LConn1 -- Controlled Current Source1/RConn2
  +/RConn1 -- Current Sensor/RConn2 -- Voltage Sensor/LConn1
  Controlled Current Source1/LConn1 -- Resistor1/RConn1 -- -/RConn1 -- Voltage Sensor/RConn2
  Simulink-PS Converter/RConn1 -- Controlled Current Source1/RConn1
  Current Sensor/RConn1 -- PS-Simulink Converter/LConn1
  PS-Simulink Converter1/LConn1 -- Voltage Sensor/RConn1

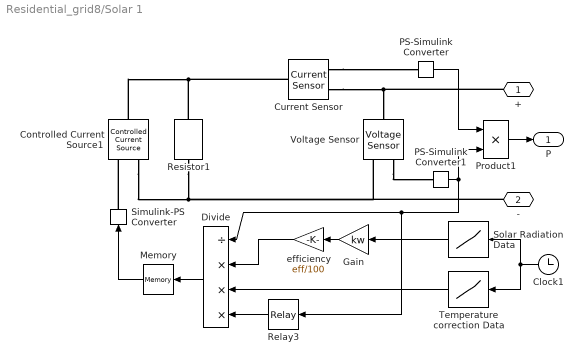
== system Residential_grid8/Solar 1 ==
  Clock1 : Clock
  Controlled Current Source1 : fl_lib/Electrical/Electrical Sources/Controlled Current Source
  Current Sensor : fl_lib/Electrical/Electrical Sensors/Current Sensor
  Divide : Product  Inputs=/***
  Gain : Gain  Gain=kw
  Memory : Memory
  PS-Simulink Converter : nesl_utility/PS-Simulink Converter  PhysicalDomain=network_engine_domain  SubClassName=ps_output  LeftPortType=input  RightPortType=output  PseudoPeriodic=off  Frequencies=[]  VectorFormat=inherit  Unit=inherit  AffineConversion=off
  PS-Simulink Converter1 : nesl_utility/PS-Simulink Converter  PhysicalDomain=network_engine_domain  SubClassName=ps_output  LeftPortType=input  RightPortType=output  PseudoPeriodic=off  Frequencies=[]  VectorFormat=inherit  Unit=inherit  AffineConversion=off
  Product1 : Product
  Relay3 : Relay  OnSwitchValue=V_stop  OffSwitchValue=V_resum  OnOutputValue=0  OffOutputValue=1
  Resistor1 : fl_lib/Electrical/Electrical Elements/Resistor  R=1e10 Ohm  i_specify=off  i_priority=None  i=0 A  i_nominal_specify=off  i_nominal_value=1  i_nominal_unit=A  v_specify=off  v_priority=None  v=0 V  v_nominal_specify=off  v_nominal_value=1  v_nominal_unit=V
  Simulink-PS Converter : nesl_utility/Simulink-PS Converter  PhysicalDomain=network_engine_domain  SubClassName=ps_input  LeftPortType=input  RightPortType=output  PseudoPeriodic=off  Frequencies=[]  NoiseDistribution=none  NoiseParameters=[]  Unit=1  AffineConversion=off  FilteringAndDerivatives=provide  SimscapeFilterOrder=1  InputFilterTimeConstant=0.001  UdotUserProvided=0
  Solar Radiation Data : Lookup_n-D  NumberOfTableDimensions=1  BreakpointsForDimension1=timestep  BeginIndexSearchUsingPreviousIndexResult=on  Table=POA  InternalRulePriority=Speed  RndMeth=Simplest
  Temperature correction Data : Lookup_n-D  NumberOfTableDimensions=1  BreakpointsForDimension1=timestep  BeginIndexSearchUsingPreviousIndexResult=on  Table=Coef  InternalRulePriority=Speed  RndMeth=Simplest
  Voltage Sensor : fl_lib/Electrical/Electrical Sensors/Voltage Sensor
  efficiency : Gain  Gain=eff/100
  + : PMIOPort  Side=Right
  - : PMIOPort  Port=2  Side=Right
  P : Outport
  wires:
  Divide/1 -> Memory/1
  Clock1/1 -> Temperature correction Data/1, Solar Radiation Data/1
  Solar Radiation Data/1 -> Gain/1
  Product1/1 -> P/1
  Gain/1 -> efficiency/1
  Memory/1 -> Simulink-PS Converter/1
  PS-Simulink Converter1/1 -> Relay3/1, Divide/1, Product1/2
  PS-Simulink Converter/1 -> Product1/1
  Temperature correction Data/1 -> Divide/3
  efficiency/1 -> Divide/2
  Relay3/1 -> Divide/4
  connections:
  Controlled Current Source1/RConn2 -- Resistor1/RConn1 -- -/RConn1 -- Voltage Sensor/RConn2
  Controlled Current Source1/LConn1 -- Current Sensor/LConn1 -- Resistor1/LConn1
  +/RConn1 -- Current Sensor/RConn2 -- Voltage Sensor/LConn1
  Current Sensor/RConn1 -- PS-Simulink Converter/LConn1
  Voltage Sensor/RConn1 -- PS-Simulink Converter1/LConn1
  Simulink-PS Converter/RConn1 -- Controlled Current Source1/RConn1

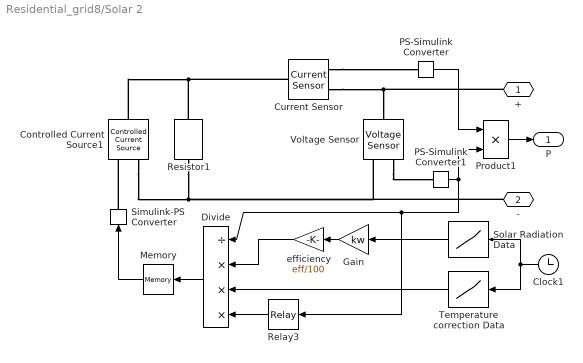
== system Residential_grid8/Solar 2 ==
  Clock1 : Clock
  Controlled Current Source1 : fl_lib/Electrical/Electrical Sources/Controlled Current Source
  Current Sensor : fl_lib/Electrical/Electrical Sensors/Current Sensor
  Divide : Product  Inputs=/***
  Gain : Gain  Gain=kw
  Memory : Memory
  PS-Simulink Converter : nesl_utility/PS-Simulink Converter  PhysicalDomain=network_engine_domain  SubClassName=ps_output  LeftPortType=input  RightPortType=output  PseudoPeriodic=off  Frequencies=[]  VectorFormat=inherit  Unit=inherit  AffineConversion=off
  PS-Simulink Converter1 : nesl_utility/PS-Simulink Converter  PhysicalDomain=network_engine_domain  SubClassName=ps_output  LeftPortType=input  RightPortType=output  PseudoPeriodic=off  Frequencies=[]  VectorFormat=inherit  Unit=inherit  AffineConversion=off
  Product1 : Product
  Relay3 : Relay  OnSwitchValue=V_stop  OffSwitchValue=V_resum  OnOutputValue=0  OffOutputValue=1
  Resistor1 : fl_lib/Electrical/Electrical Elements/Resistor  R=1e10 Ohm  i_specify=off  i_priority=None  i=0 A  i_nominal_specify=off  i_nominal_value=1  i_nominal_unit=A  v_specify=off  v_priority=None  v=0 V  v_nominal_specify=off  v_nominal_value=1  v_nominal_unit=V
  Simulink-PS Converter : nesl_utility/Simulink-PS Converter  PhysicalDomain=network_engine_domain  SubClassName=ps_input  LeftPortType=input  RightPortType=output  PseudoPeriodic=off  Frequencies=[]  NoiseDistribution=none  NoiseParameters=[]  Unit=1  AffineConversion=off  FilteringAndDerivatives=provide  SimscapeFilterOrder=1  InputFilterTimeConstant=0.001  UdotUserProvided=0
  Solar Radiation Data : Lookup_n-D  NumberOfTableDimensions=1  BreakpointsForDimension1=timestep  BeginIndexSearchUsingPreviousIndexResult=on  Table=POA  InternalRulePriority=Speed  RndMeth=Simplest
  Temperature correction Data : Lookup_n-D  NumberOfTableDimensions=1  BreakpointsForDimension1=timestep  BeginIndexSearchUsingPreviousIndexResult=on  Table=Coef  InternalRulePriority=Speed  RndMeth=Simplest
  Voltage Sensor : fl_lib/Electrical/Electrical Sensors/Voltage Sensor
  efficiency : Gain  Gain=eff/100
  + : PMIOPort  Side=Right
  - : PMIOPort  Port=2  Side=Right
  P : Outport
  wires:
  Divide/1 -> Memory/1
  Clock1/1 -> Temperature correction Data/1, Solar Radiation Data/1
  Solar Radiation Data/1 -> Gain/1
  Product1/1 -> P/1
  Gain/1 -> efficiency/1
  Memory/1 -> Simulink-PS Converter/1
  PS-Simulink Converter1/1 -> Relay3/1, Divide/1, Product1/2
  PS-Simulink Converter/1 -> Product1/1
  Temperature correction Data/1 -> Divide/3
  efficiency/1 -> Divide/2
  Relay3/1 -> Divide/4
  connections:
  Controlled Current Source1/RConn2 -- Resistor1/RConn1 -- -/RConn1 -- Voltage Sensor/RConn2
  Controlled Current Source1/LConn1 -- Current Sensor/LConn1 -- Resistor1/LConn1
  +/RConn1 -- Current Sensor/RConn2 -- Voltage Sensor/LConn1
  Current Sensor/RConn1 -- PS-Simulink Converter/LConn1
  Voltage Sensor/RConn1 -- PS-Simulink Converter1/LConn1
  Simulink-PS Converter/RConn1 -- Controlled Current Source1/RConn1
